simulink subsystem "DC7960MDriver"  (R2026a)
settings: Solver=VariableStepAuto
libraries: arduinolib x4
settings Model: Creator=bence  LastModifiedBy=bence

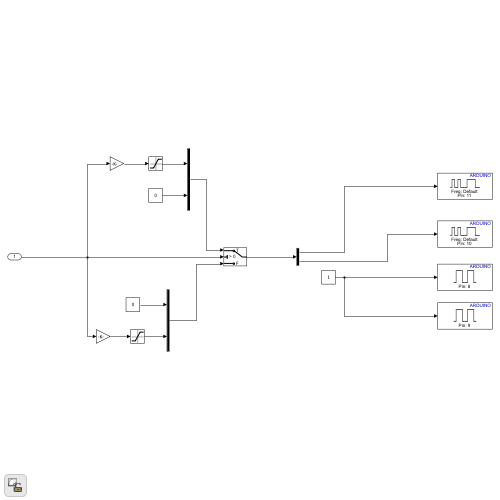
[thumbnail: Simulink's stored preview of the top-level diagram]
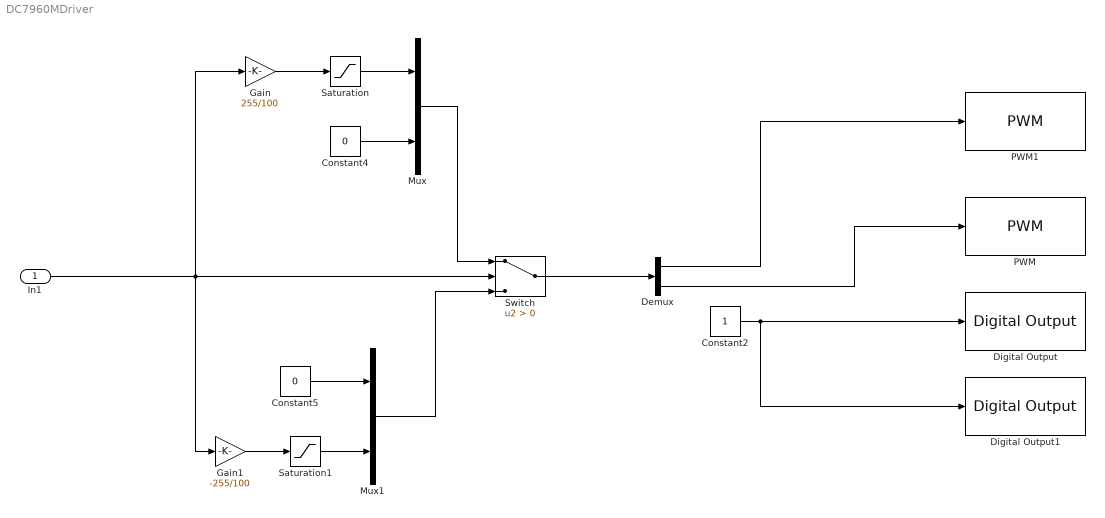
== system DC7960MDriver ==
  In1 : Inport
  Constant2 : Constant  OutDataTypeStr=single
  Constant4 : Constant  Value=0  OutDataTypeStr=single
  Constant5 : Constant  Value=0  OutDataTypeStr=single
  Demux : Demux  Outputs=2
  Digital Output : arduinolib/Digital Output  pinNumber=8  Direction=output  blockPlatform=arduino
  Digital Output1 : arduinolib/Digital Output  pinNumber=9  Direction=output  blockPlatform=arduino
  Gain : Gain  Gain=255/100  OutDataTypeStr=single
  Gain1 : Gain  Gain=-255/100  OutDataTypeStr=single
  Mux : Mux  Inputs=2
  Mux1 : Mux  Inputs=2
  PWM : arduinolib/PWM  pinNumber=10  frequencyType=Default  desiredFrequency=490.2  achievableFrequency=490.2
  PWM1 : arduinolib/PWM  pinNumber=11  frequencyType=Default  desiredFrequency=490.2  achievableFrequency=490.2
  Saturation : Saturate  UpperLimit=255  LowerLimit=0
  Saturation1 : Saturate  UpperLimit=255  LowerLimit=0
  Switch : Switch  Criteria=u2 > Threshold  OutDataTypeStr=single  SaturateOnIntegerOverflow=off  InputSameDT=off
  wires:
  Mux1/1 -> Switch/3
  Switch/1 -> Demux/1
  Gain/1 -> Saturation/1
  Saturation/1 -> Mux/1
  In1/1 -> Switch/2, Gain/1, Gain1/1
  Constant2/1 -> Digital Output/1, Digital Output1/1
  Demux/1 -> PWM1/1
  Constant5/1 -> Mux1/1
  Constant4/1 -> Mux/2
  Mux/1 -> Switch/1
  Gain1/1 -> Saturation1/1
  Demux/2 -> PWM/1
  Saturation1/1 -> Mux1/2
